simulink model "PassivityBasedFinale"  (R2024b)
settings: Solver=VariableStepAuto  StartTime=0.0  StopTime=60  RelTol=1e-3
InitFcn:
  | %  Butterworth filter
  |  r=3;
  |  [b, a] = butter(r, 5, 'low', 's');  % Butterworth filter of order r
  |  K = zeros(r,1);
  |  prod = 1;
  |  for j = 1:r
  |      K(j) = a(j+1)/prod;
  |     prod = prod*K(j);
  |  end
  |  K = flip(K);
  | 
  |  intv=[];
  |  for i=1:r
  |     v(i).vec = zeros(6,1);
  |      intv = [intv,v(i).vec];
  |  end
values from neighbouring files (symbols this model uses):
  Ts = 0.001    [traj_genPassivity.m]
undefined symbols (not defined in the file or in its folder): dspblkCoreblockFVToolHelper, gcbh
libraries: robotcorelib x1, uavutilslib x1
settings Model: Creator=mattr  LastModifiedBy=mattr

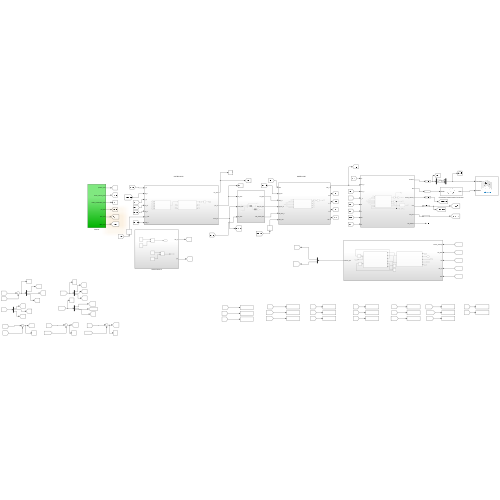
[thumbnail: Simulink's stored preview of the top-level diagram]
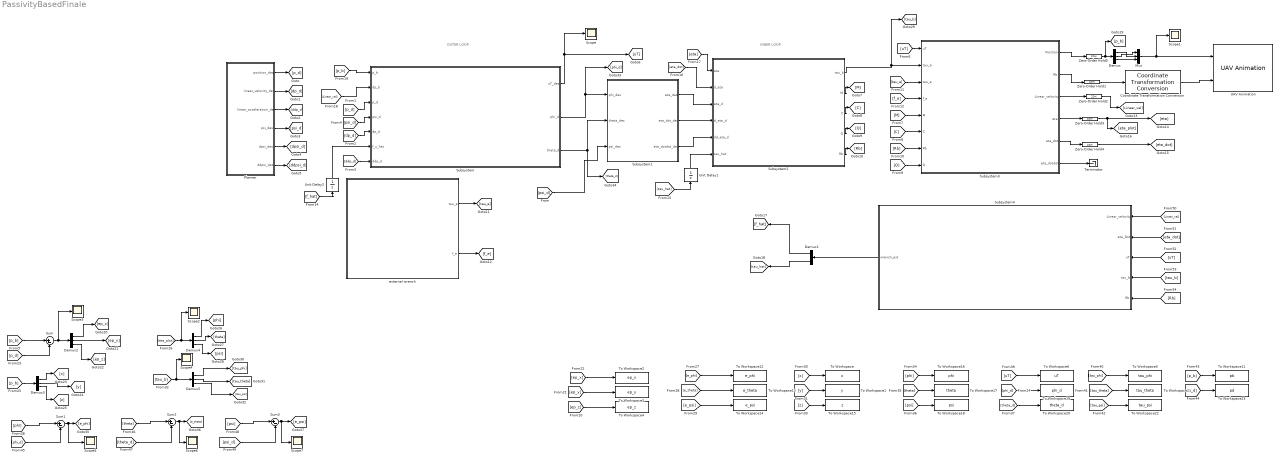
== system PassivityBasedFinale ==
  note: INNER LOOP
  note: OUTER LOOP
  Coordinate Transformation Conversion : robotcorelib/Coordinate Transformation Conversion  InputRepresentation=Rotation Matrix  InputEulerSequence=ZYX  ShowTrVecInputPort=on  OutputRepresentation=Quaternion  OutputEulerSequence=ZYX  ShowTrVecOutputPort=on  SimulateUsing=Interpreted execution
  Demux{,2..5} (5 alike) : Demux  Outputs=3
  Demux1 : Demux  Outputs=2
  Mux : Mux  Inputs=3
  Planner : Subsystem
  Scope{,1..7} (8 alike) : Scope
  Subsystem : Subsystem
  Subsystem1 : Subsystem
  Subsystem2 : Subsystem
  Subsystem3 : Subsystem
  Subsystem4 : Subsystem
  Sum{,1..3} (4 alike) : Sum  Inputs=|+-
  Terminator : Terminator
  To Workspace : ToWorkspace  VariableName=x  SaveFormat=Timeseries  SampleTime=-1
  To Workspace1 : ToWorkspace  VariableName=y  SaveFormat=Timeseries  SampleTime=-1
  To Workspace11 : ToWorkspace  VariableName=pb  SaveFormat=Timeseries  SampleTime=-1
  To Workspace12 : ToWorkspace  VariableName=e_phi  SaveFormat=Timeseries  SampleTime=-1
  To Workspace13 : ToWorkspace  VariableName=e_theta  SaveFormat=Timeseries  SampleTime=-1
  To Workspace14 : ToWorkspace  VariableName=e_psi  SaveFormat=Timeseries  SampleTime=-1
  To Workspace15 : ToWorkspace  VariableName=z  SaveFormat=Timeseries  SampleTime=-1
  To Workspace16 : ToWorkspace  VariableName=phi  SaveFormat=Timeseries  SampleTime=-1
  To Workspace17 : ToWorkspace  VariableName=theta  SaveFormat=Timeseries  SampleTime=-1
  To Workspace18 : ToWorkspace  VariableName=psi  SaveFormat=Timeseries  SampleTime=-1
  To Workspace19 : ToWorkspace  VariableName=phi_d  SaveFormat=Timeseries  SampleTime=-1
  To Workspace2 : ToWorkspace  VariableName=ep_x  SaveFormat=Timeseries  SampleTime=-1
  To Workspace20 : ToWorkspace  VariableName=theta_d  SaveFormat=Timeseries  SampleTime=-1
  To Workspace21 : ToWorkspace  VariableName=tau_theta  SaveFormat=Timeseries  SampleTime=-1
  To Workspace22 : ToWorkspace  VariableName=tau_psi  SaveFormat=Timeseries  SampleTime=-1
  To Workspace23 : ToWorkspace  VariableName=pd  SaveFormat=Timeseries  SampleTime=-1
  To Workspace3 : ToWorkspace  VariableName=ep_y  SaveFormat=Timeseries  SampleTime=-1
  To Workspace4 : ToWorkspace  VariableName=ep_z  SaveFormat=Timeseries  SampleTime=-1
  To Workspace5 : ToWorkspace  VariableName=tau_phi  SaveFormat=Timeseries  SampleTime=-1
  To Workspace6 : ToWorkspace  VariableName=uT  SaveFormat=Timeseries  SampleTime=-1
  UAV Animation : uavutilslib/UAV Animation  NumUAV=1  DynamicUAVConfig=off  UAVType=Multirotor  UAVSize=1  UAVColor=[1 0 0]  UAVTrajectoryAlpha=1  InertialZDirection=Up  RotationFormat=Quaternion  DrawMarkers=off  SampleTime=-1
  Unit Delay1 : UnitDelay  InitialCondition=Ts  SampleTime=-1  HasFrameUpgradeWarning=on
  Unit Delay2 : UnitDelay  InitialCondition=Ts  SampleTime=-1  HasFrameUpgradeWarning=on
  Zero-Order Hold{1..5} (5 alike) : ZeroOrderHold  SampleTime=Ts
  external wrench : Subsystem
  wires:
  Planner/1(position_des) -> [p_d]
  [p_d] -> Subsystem/3(p_d)
  Planner/2(linear_velocity_des) -> [dp_d]
  [dp_d] -> Subsystem/5(dp_d)
  Planner/3(linear_acceleration_des) -> [ddp_d]
  [ddp_d] -> Subsystem/7(ddp_d)
  Planner/4(psi_des) -> [psi_d]
  [psi_d] -> Subsystem/4(psi_d)
  Planner/5(dpsi_des) -> [dpsi_d]
  Planner/6(ddpsi_des) -> [ddpsi_d]
  Subsystem/2(phi_d) -> Subsystem1/1(phi_des), [phi_d]
  Subsystem/3(theta_d) -> [theta_d], Subsystem1/2(theta_des)
  [psi_d] -> Subsystem1/3(psi_des)
  Subsystem1/1(eta_des) -> Subsystem2/3(eta_d)
  Subsystem1/2(eta_dot_des) -> Subsystem2/4(d_eta_d)
  Subsystem1/3(eta_dotdot_des) -> Subsystem2/5(dd_eta_d)
  [uT] -> Subsystem3/1(uT)
  Subsystem2/1(tau_b) -> [tau_b], Subsystem3/2(tau_b)
  Subsystem2/3(C) -> [C]
  Subsystem2/2(M) -> [M]
  Subsystem2/4(Q) -> [Q]
  Subsystem2/5(Rb) -> [Rb]
  [M] -> Subsystem3/5(M)
  [C] -> Subsystem3/6(C)
  [Q] -> Subsystem3/8(Q)
  [Rb] -> Subsystem3/7("Rb ")
  [tau_e] -> Subsystem3/3(tau_e)
  [f_e] -> Subsystem3/4(f_e)
  external wrench/2(f_e) -> [f_e]
  external wrench/1(tau_e) -> [tau_e]
  Zero-Order Hold1/1 -> Coordinate Transformation Conversion/1
  Coordinate Transformation Conversion/1 -> UAV Animation/2
  Subsystem3/1(Position) -> Zero-Order Hold5/1
  Zero-Order Hold5/1 -> [p_b], Demux/1
  Demux/1 -> Mux/2
  Demux/2 -> Mux/1
  Demux/3 -> Mux/3
  Mux/1 -> Scope1/1, UAV Animation/1
  Zero-Order Hold2/1 -> [Linear_vel]
  Zero-Order Hold3/1 -> [eta_plot], [eta]
  Subsystem3/6(eta_dotdot) -> Terminator/1
  Zero-Order Hold4/1 -> [eta_dot]
  Subsystem4/1(wrench_ext) -> Demux1/1
  Demux1/1 -> [f_hat]
  Demux1/2 -> [tau_hat]
  [f_hat] -> Unit Delay2/1
  [tau_hat] -> Unit Delay1/1
  Unit Delay1/1 -> Subsystem2/6(tau_hat)
  [eta] -> Subsystem2/1(eta)
  [eta_dot] -> Subsystem2/2(d_eta)
  [p_b] -> Subsystem/1(p_b)
  [Linear_vel] -> Subsystem/2(dp_b)
  [theta] -> To Workspace17/1
  [x] -> To Workspace/1
  [p_b] -> To Workspace11/1
  [ep_x] -> To Workspace2/1
  [e_psi] -> To Workspace14/1
  [ep_y] -> To Workspace3/1
  [theta_d] -> To Workspace20/1
  [psi] -> To Workspace18/1
  [tau_psi] -> To Workspace22/1
  [e_phi] -> To Workspace12/1
  [tau_theta] -> To Workspace21/1
  [p_d] -> To Workspace23/1
  [y] -> To Workspace1/1
  [z] -> To Workspace15/1
  [phi_d] -> To Workspace19/1
  [e_theta] -> To Workspace13/1
  [uT] -> To Workspace6/1
  [tau_phi] -> To Workspace5/1
  [phi] -> To Workspace16/1
  [ep_z] -> To Workspace4/1
  [p_b] -> Sum/1
  [p_d] -> Sum/2
  Sum/1 -> Scope3/1, Demux2/1
  Demux2/1 -> [ep_x]
  Demux2/2 -> [ep_y]
  Demux2/3 -> [ep_z]
  [p_b] -> Demux3/1
  Demux3/1 -> [x]
  Demux3/2 -> [y]
  Demux3/3 -> [z]
  [eta_plot] -> Scope2/1, Demux4/1
  Demux4/1 -> [phi]
  Demux4/2 -> [theta]
  Demux4/3 -> [psi]
  [tau_b] -> Scope4/1, Demux5/1
  Demux5/1 -> [tau_phi]
  Demux5/2 -> [tau_theta]
  Demux5/3 -> [tau_psi]
  [phi] -> Sum1/1
  [phi_d] -> Sum1/2
  Sum1/1 -> Scope5/1, [e_phi]
  [theta] -> Sum2/1
  [theta_d] -> Sum2/2
  Sum2/1 -> Scope6/1, [e_theta]
  Sum3/1 -> Scope7/1, [e_psi]
  [psi] -> Sum3/1
  [psi_d] -> Sum3/2
  Subsystem/1(uT_des) -> [uT], Scope/1
  [Linear_vel] -> Subsystem4/1(Linear_velocity)
  [eta_dot] -> Subsystem4/2(eta_Dot)
  [uT] -> Subsystem4/3(uT)
  [tau_b] -> Subsystem4/4(tau_b)
  [Rb] -> Subsystem4/5(Rb)
  Unit Delay2/1 -> Subsystem/6(f_u_hat)
  Subsystem3/2(Rb) -> Zero-Order Hold1/1
  Subsystem3/3(Linear_velocity) -> Zero-Order Hold2/1
  Subsystem3/4(eta) -> Zero-Order Hold3/1
  Subsystem3/5(eta_dot) -> Zero-Order Hold4/1

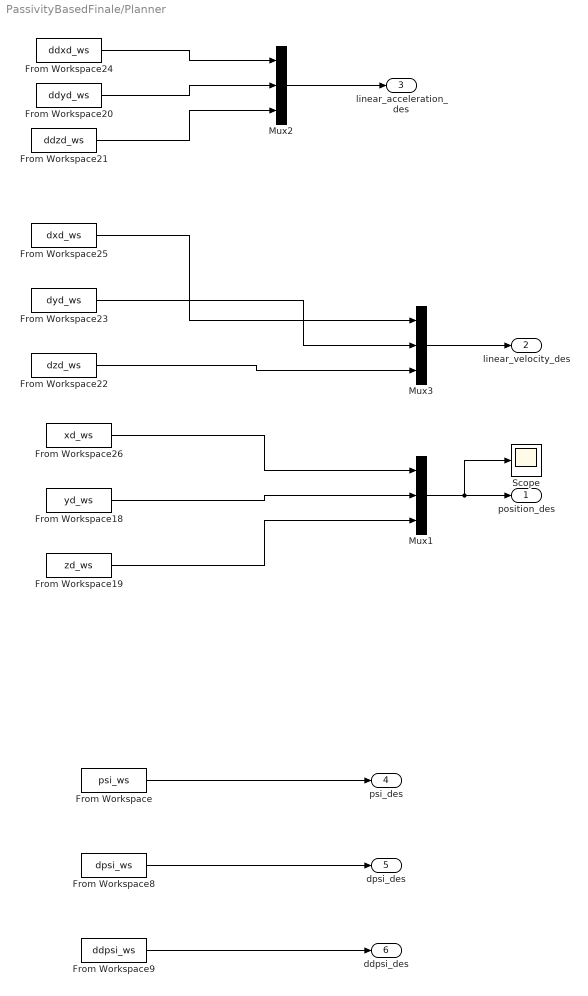
== system PassivityBasedFinale/Planner ==
  From Workspace : FromWorkspace  VariableName=psi_ws
  From Workspace18 : FromWorkspace  VariableName=yd_ws
  From Workspace19 : FromWorkspace  VariableName=zd_ws
  From Workspace20 : FromWorkspace  VariableName=ddyd_ws
  From Workspace21 : FromWorkspace  VariableName=ddzd_ws
  From Workspace22 : FromWorkspace  VariableName=dzd_ws
  From Workspace23 : FromWorkspace  VariableName=dyd_ws
  From Workspace24 : FromWorkspace  VariableName=ddxd_ws
  From Workspace25 : FromWorkspace  VariableName=dxd_ws
  From Workspace26 : FromWorkspace  VariableName=xd_ws
  From Workspace8 : FromWorkspace  VariableName=dpsi_ws
  From Workspace9 : FromWorkspace  VariableName=ddpsi_ws
  Mux1 : Mux  Inputs=3
  Mux2 : Mux  Inputs=3
  Mux3 : Mux  Inputs=3
  Scope : Scope
  position_des : Outport
  linear_velocity_des : Outport  Port=2
  linear_acceleration_des : Outport  Port=3
  psi_des : Outport  Port=4
  dpsi_des : Outport  Port=5
  ddpsi_des : Outport  Port=6
  wires:
  Mux2/1 -> linear_acceleration_des/1
  Mux1/1 -> Scope/1, position_des/1
  Mux3/1 -> linear_velocity_des/1
  From Workspace26/1 -> Mux1/1
  From Workspace18/1 -> Mux1/2
  From Workspace19/1 -> Mux1/3
  From Workspace25/1 -> Mux3/1
  From Workspace23/1 -> Mux3/2
  From Workspace22/1 -> Mux3/3
  From Workspace24/1 -> Mux2/1
  From Workspace20/1 -> Mux2/2
  From Workspace21/1 -> Mux2/3
  From Workspace/1 -> psi_des/1
  From Workspace8/1 -> dpsi_des/1
  From Workspace9/1 -> ddpsi_des/1

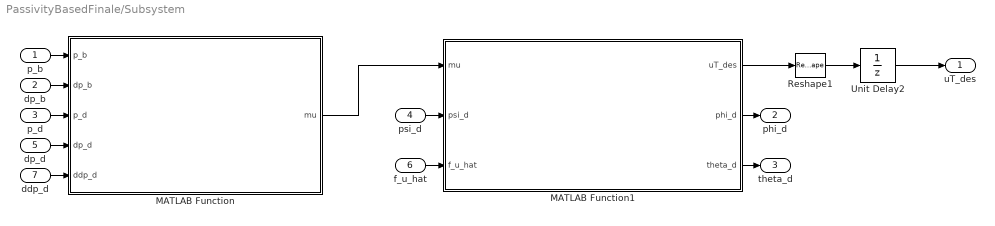
== system PassivityBasedFinale/Subsystem ==
  p_b : Inport
  dp_b : Inport  Port=2
  p_d : Inport  Port=3
  psi_d : Inport  Port=4
  dp_d : Inport  Port=5
  f_u_hat : Inport  Port=6
  ddp_d : Inport  Port=7
  MATLAB Function : MATLAB Function  TreatAsAtomicUnit=on
  MATLAB Function1 : MATLAB Function  TreatAsAtomicUnit=on
  Reshape1 : Reshape
  Unit Delay2 : UnitDelay  InitialCondition=12  SampleTime=Ts  HasFrameUpgradeWarning=on
  uT_des : Outport
  phi_d : Outport  Port=2
  theta_d : Outport  Port=3
  wires:
  p_b/1 -> MATLAB Function/1(p_b)
  psi_d/1 -> MATLAB Function1/2(psi_d)
  ddp_d/1 -> MATLAB Function/5(ddp_d)
  f_u_hat/1 -> MATLAB Function1/3(f_u_hat)
  dp_d/1 -> MATLAB Function/4(dp_d)
  dp_b/1 -> MATLAB Function/2(dp_b)
  p_d/1 -> MATLAB Function/3(p_d)
  MATLAB Function1/2(phi_d) -> phi_d/1
  MATLAB Function1/3(theta_d) -> theta_d/1
  MATLAB Function1/1(uT_des) -> Reshape1/1
  Reshape1/1 -> Unit Delay2/1
  Unit Delay2/1 -> uT_des/1
  MATLAB Function/1(mu) -> MATLAB Function1/1(mu)

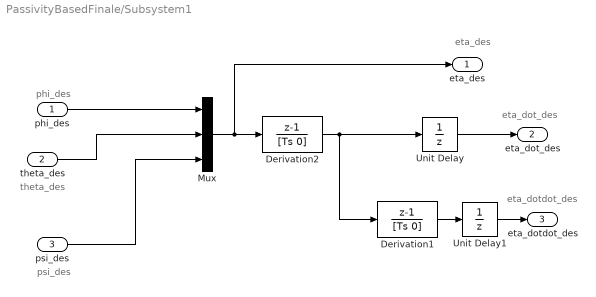
== system PassivityBasedFinale/Subsystem1 ==
  note: eta_dotdot_des
  note: eta_dot_des
  note: eta_des
  note: theta_des
  note: psi_des
  note: phi_des
  phi_des : Inport
  theta_des : Inport  Port=2
  psi_des : Inport  Port=3
  Derivation1 : DiscreteTransferFcn  LoadFcn=dspblkCoreblockFVToolHelper(gcbh,'load');  Numerator=[1 -1]  Denominator=[Ts 0]  InitialStates=[0 0 0]  SampleTime=Ts
      settings: CopyFcn=dspblkCoreblockFVToolHelper(gcbh,'copy');  DeleteFcn=dspblkCoreblockFVToolHelper(gcbh,'close');  ModelCloseFcn=dspblkCoreblockFVToolHelper(gcbh,'close');  PreSaveFcn=dspblkCoreblockFVToolHelper(gcbh,'presave');  PostSaveFcn=dspblkCoreblockFVToolHelper(gcbh,'postsave');  CloseFcn=dspblkCoreblockFVToolHelper(gcbh,'close');
  Derivation2 : DiscreteTransferFcn  LoadFcn=dspblkCoreblockFVToolHelper(gcbh,'load');  Numerator=[1 -1]  Denominator=[Ts 0]  InitialStates=[0 0 0]  SampleTime=Ts
      settings: CopyFcn=dspblkCoreblockFVToolHelper(gcbh,'copy');  DeleteFcn=dspblkCoreblockFVToolHelper(gcbh,'close');  ModelCloseFcn=dspblkCoreblockFVToolHelper(gcbh,'close');  PreSaveFcn=dspblkCoreblockFVToolHelper(gcbh,'presave');  PostSaveFcn=dspblkCoreblockFVToolHelper(gcbh,'postsave');  CloseFcn=dspblkCoreblockFVToolHelper(gcbh,'close');
  Mux : Mux  Inputs=3
  Unit Delay : UnitDelay  InitialCondition=[0 0 0]  SampleTime=-1  HasFrameUpgradeWarning=on
  Unit Delay1 : UnitDelay  InitialCondition=[0 0 0]  SampleTime=-1  HasFrameUpgradeWarning=on
  eta_des : Outport
  eta_dot_des : Outport  Port=2
  eta_dotdot_des : Outport  Port=3
  wires:
  psi_des/1 -> Mux/3
  theta_des/1 -> Mux/2
  phi_des/1 -> Mux/1
  Mux/1 -> Derivation2/1, eta_des/1
  Derivation2/1 -> Derivation1/1, Unit Delay/1
  Unit Delay/1 -> eta_dot_des/1
  Derivation1/1 -> Unit Delay1/1
  Unit Delay1/1 -> eta_dotdot_des/1

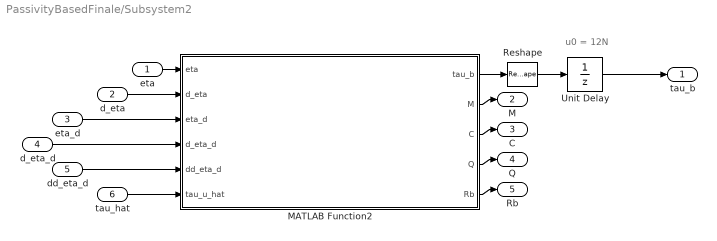
== system PassivityBasedFinale/Subsystem2 ==
  note: u0 = 12N
  eta : Inport
  d_eta : Inport  Port=2
  eta_d : Inport  Port=3
  d_eta_d : Inport  Port=4
  dd_eta_d : Inport  Port=5
  tau_hat : Inport  Port=6
  MATLAB Function2 : MATLAB Function  TreatAsAtomicUnit=on
  Reshape : Reshape
  Unit Delay : UnitDelay  InitialCondition=12  SampleTime=Ts  HasFrameUpgradeWarning=on
  tau_b : Outport
  M : Outport  Port=2
  C : Outport  Port=3
  Q : Outport  Port=4
  Rb : Outport  Port=5
  wires:
  d_eta/1 -> MATLAB Function2/2(d_eta)
  MATLAB Function2/4(Q) -> Q/1
  MATLAB Function2/3(C) -> C/1
  d_eta_d/1 -> MATLAB Function2/4(d_eta_d)
  dd_eta_d/1 -> MATLAB Function2/5(dd_eta_d)
  eta/1 -> MATLAB Function2/1(eta)
  MATLAB Function2/2(M) -> M/1
  eta_d/1 -> MATLAB Function2/3(eta_d)
  MATLAB Function2/5(Rb) -> Rb/1
  tau_hat/1 -> MATLAB Function2/6(tau_u_hat)
  Reshape/1 -> Unit Delay/1
  MATLAB Function2/1(tau_b) -> Reshape/1
  Unit Delay/1 -> tau_b/1

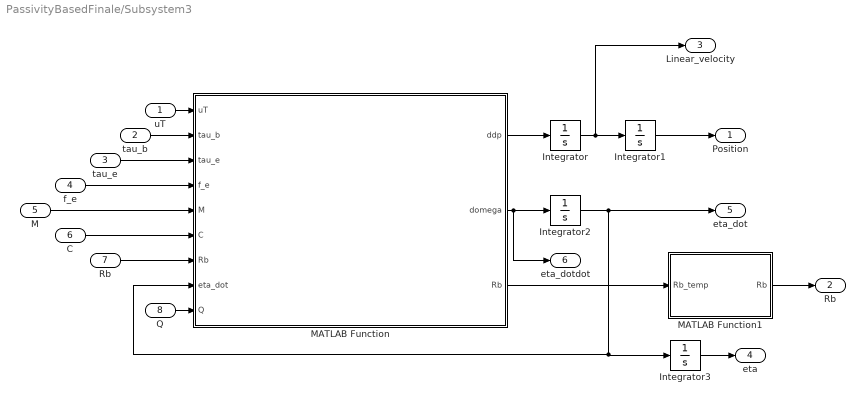
== system PassivityBasedFinale/Subsystem3 ==
  uT : Inport
  tau_b : Inport  Port=2
  tau_e : Inport  Port=3
  f_e : Inport  Port=4
  M : Inport  Port=5
  C : Inport  Port=6
  "Rb " : Inport  Port=7
  Q : Inport  Port=8
  Integrator : Integrator  InitialCondition=|
      | [ -9.8696e-05, 
      |     0.6283
      | ,    3.3333e-06]
  Integrator1 : Integrator  InitialCondition=[0 0 0]
  Integrator2 : Integrator  InitialCondition=[0 0 0]'
  Integrator3 : Integrator  InitialCondition=[0 0 0]'
  MATLAB Function : MATLAB Function  TreatAsAtomicUnit=on
  MATLAB Function1 : MATLAB Function  TreatAsAtomicUnit=on
  Position : Outport
  Rb : Outport  Port=2
  Linear_velocity : Outport  Port=3
  eta : Outport  Port=4
  eta_dot : Outport  Port=5
  eta_dotdot : Outport  Port=6
  wires:
  C/1 -> MATLAB Function/6(C)
  "Rb "/1 -> MATLAB Function/7("Rb ")
  tau_e/1 -> MATLAB Function/3(tau_e)
  tau_b/1 -> MATLAB Function/2(tau_b)
  f_e/1 -> MATLAB Function/4(f_e)
  uT/1 -> MATLAB Function/1(uT)
  M/1 -> MATLAB Function/5(M)
  Q/1 -> MATLAB Function/9(Q)
  MATLAB Function/3(Rb) -> MATLAB Function1/1(Rb_temp)
  MATLAB Function/1(ddp) -> Integrator/1
  Integrator/1 -> Linear_velocity/1, Integrator1/1
  Integrator1/1 -> Position/1
  MATLAB Function/2(domega) -> eta_dotdot/1, Integrator2/1
  Integrator2/1 -> MATLAB Function/8(eta_dot), Integrator3/1, eta_dot/1
  MATLAB Function1/1(Rb) -> Rb/1
  Integrator3/1 -> eta/1

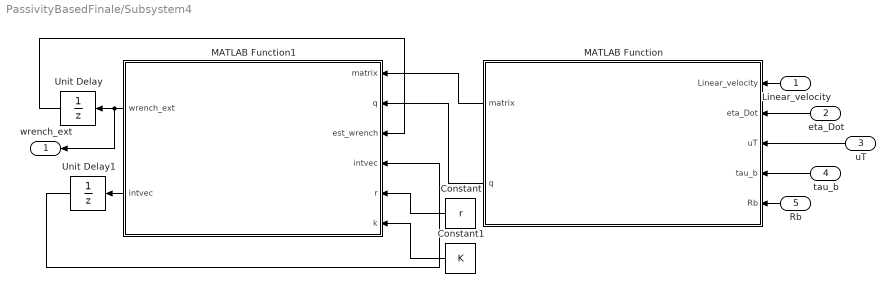
== system PassivityBasedFinale/Subsystem4 ==
  Linear_velocity : Inport
  eta_Dot : Inport  Port=2
  uT : Inport  Port=3
  tau_b : Inport  Port=4
  Rb : Inport  Port=5
  Constant : Constant  Value=r
  Constant1 : Constant  Value=K
  MATLAB Function : MATLAB Function  TreatAsAtomicUnit=on
  MATLAB Function1 : MATLAB Function  TreatAsAtomicUnit=on
  Unit Delay : UnitDelay  InitialCondition=zeros(6,1)  SampleTime=Ts  HasFrameUpgradeWarning=on
  Unit Delay1 : UnitDelay  InitialCondition=intv  SampleTime=Ts  HasFrameUpgradeWarning=on
  wrench_ext : Outport
  wires:
  Constant/1 -> MATLAB Function1/5(r)
  Unit Delay1/1 -> MATLAB Function1/4("intvec ")
  MATLAB Function1/2(intvec) -> Unit Delay1/1
  MATLAB Function/2(q) -> MATLAB Function1/2(q)
  Linear_velocity/1 -> MATLAB Function/1(Linear_velocity)
  tau_b/1 -> MATLAB Function/4(tau_b)
  uT/1 -> MATLAB Function/3(uT)
  Rb/1 -> MATLAB Function/5(Rb)
  eta_Dot/1 -> MATLAB Function/2(eta_Dot)
  MATLAB Function/1(matrix) -> MATLAB Function1/1(matrix)
  Unit Delay/1 -> MATLAB Function1/3(est_wrench)
  Constant1/1 -> MATLAB Function1/6(k)
  MATLAB Function1/1(wrench_ext) -> wrench_ext/1, Unit Delay/1

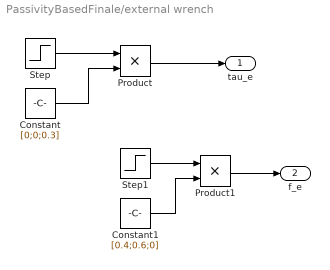
== system PassivityBasedFinale/external wrench ==
  Constant : Constant  Value=[0;0;0.3]  SampleTime=Ts
  Constant1 : Constant  Value=[0.4;0.6;0]  SampleTime=Ts
  Product : Product
  Product1 : Product
  Step : Step  Time=12  SampleTime=Ts
  Step1 : Step  Time=12  SampleTime=Ts
  tau_e : Outport
  f_e : Outport  Port=2
  wires:
  Step1/1 -> Product1/1
  Constant/1 -> Product/2
  Constant1/1 -> Product1/2
  Step/1 -> Product/1
  Product1/1 -> f_e/1
  Product/1 -> tau_e/1

== matlab function PassivityBasedFinale/Subsystem/MATLAB Function1 ==
  data: mu input; uT_des output; psi_d input; f_u_hat input; phi_d output; theta_d output
function [uT_des, phi_d,theta_d] = thrust_attitude_ref(mu, psi_d, f_u_hat)
% === PARAMETERS ===
m = 1.8;
g = 9.81;

mu_bar = mu - (1/m) * f_u_hat;
mu1 = mu_bar(1);
mu2 = mu_bar(2);
mu3 = mu_bar(3);

% === THRUST ===
uT_des = m * sqrt(mu1^2 + mu2^2 + (mu3 - g)^2);

% === DESIRED ANGLES ===
phi_arg = (m/uT_des)*(mu2 * cos(psi_d) - mu1 * sin(psi_d));
phi_d = asin(phi_arg);
theta_d = atan((mu1 * cos(psi_d) + mu2 * sin(psi_d))/(mu3 - g));
end

== matlab function PassivityBasedFinale/Subsystem/MATLAB Function ==
  data: p_b input; mu output; dp_b input; p_d input; dp_d input; ddp_d input
function mu = position_passive_control(p_b, dp_b, ...
                                        p_d, dp_d, ddp_d)
m = 1.8;

Kp = diag([25, 25, 10]);
Dp = diag([10, 10, 20]);

e_p = p_b - p_d;
de_p = dp_b - dp_d;

mu = ddp_d - (1/m)*(Dp*de_p + Kp*e_p);
end

== matlab function PassivityBasedFinale/Subsystem2/MATLAB Function2 ==
  data: eta input; tau_b output; d_eta input; eta_d input; d_eta_d input; dd_eta_d input; M output; C output; Q output; Rb output; tau_u_hat input
function [tau_b, M,C,Q,Rb] = attitude_passive_control(eta, d_eta, ...
    eta_d, d_eta_d, dd_eta_d, ...
    tau_u_hat)
% === PARAMETERS ===
Ko = diag([36, 36, 90]);
Do = diag([4, 4, 16]);
nu = 2; % Coupling parameter 

% Drone inertia
I = diag([0.035, 0.035, 0.05]); % Inertia matrix [kg·m²]

% === TRACKING ERRORS ===
e_eta = eta - eta_d; % angular position error
de_eta = d_eta - d_eta_d; % angular velocity error

% === REFERENCE VELOCITY  ===
d_eta_r = d_eta_d - nu * e_eta; % η̇_r = η̇_d - ν*e_η

% === REFERENCE ACCELERATION ===
dd_eta_r = dd_eta_d - nu * de_eta; % η̈_r = η̈_d - ν*ė_η

% === VELOCITY ERROR v_η  ===
v_eta = de_eta + nu * e_eta; % v_η = ė_η + ν*e_η


phi = eta(1);
theta = eta(2);
psi = eta(3);

c_phi = cos(phi); s_phi = sin(phi);
c_theta = cos(theta); s_theta = sin(theta);

Q = [1, 0, -s_theta;
     0, c_phi, s_phi*c_theta;
     0, -s_phi, c_phi*c_theta];

M = Q' * I * Q;

dphi = d_eta(1);
dtheta = d_eta(2);
dpsi = d_eta(3);

dQ = [0, 0, -c_theta*dtheta;
      0, -s_phi*dphi, c_phi*c_theta*dphi - s_phi*s_theta*dtheta;
      0, -c_phi*dphi, +s_phi*c_theta*dphi - c_phi*s_theta*dtheta];

omega_b = Q * d_eta; % angular velocity in body frame
S_omega_b = skew(omega_b);
C = Q' * S_omega_b * I * Q + Q' * I * dQ;

Rb = [cos(psi)*cos(theta), -sin(psi)*cos(phi)+cos(psi)*sin(theta)*sin(phi), sin(psi)*sin(phi)+cos(psi)*sin(theta)*cos(phi);
      sin(psi)*cos(theta), cos(psi)*cos(phi)+sin(psi)*sin(theta)*sin(phi), -cos(psi)*sin(phi)+sin(psi)*sin(theta)*cos(phi);
      -sin(theta), cos(theta)*sin(phi), cos(theta)*cos(phi)];

% Controller term
control_term = M * dd_eta_r + C * d_eta_r - Do * v_eta - Ko * e_eta - tau_u_hat;
tau_b = Q' \ control_term;
end

% === SKEW MATRIX ===
function S = skew(v)
if length(v) == 3
    S = [ 0   -v(3)  v(2);
         v(3)   0   -v(1);
        -v(2)  v(1)   0  ];
else
    S = zeros(3,3);
end
end

== matlab function PassivityBasedFinale/Subsystem3/MATLAB Function ==
  data: uT input; ddp output; tau_b input; tau_e input; f_e input; M input; C input; Rb input; eta_dot input; Q input; domega output; Rb output
function [ddp,domega,Rb]=vtol_uav(uT,tau_b,tau_e,f_e,M,C,Rb,eta_dot,Q)
% === PARAMETERS ===
mass = 1.8; % mass [kg]
g = 9.81; % gravity [m/s²]


% === TRANSLATIONAL DYNAMICS ===
ddp = 9.81*[0 0 1]' - (uT/mass)*Rb*[0 0 1]' + (1/mass)*f_e;

% === ROTATIONAL DYNAMICS ===
domega = M\(-C*eta_dot + Q'*tau_b + tau_e);
end

== matlab function PassivityBasedFinale/Subsystem3/MATLAB Function1 ==
  data: Rb_temp input; Rb output
function Rb = fcn(Rb_temp)
    [U,S,V] = svd(Rb_temp);
    sigma = det(U*V');
    S_ = diag([1 1 sigma]);

    Rb = U*S_*V';
end

== matlab function PassivityBasedFinale/Subsystem4/MATLAB Function ==
  data: Linear_velocity input; matrix output; eta_Dot input; uT input; tau_b input; Rb input; q output
function [matrix, q] = computations(Linear_velocity, eta_Dot, uT, tau_b, Rb)
mass= 1.8; 
g = 9.81;
Ib = diag([0.035, 0.035, 0.05]);
q = [mass*eye(3) zeros(3); zeros(3) Ib] * [Linear_velocity; eta_Dot];  
matrix = [mass*g*[0 0 1]'-uT*Rb*[0 0 1]'; -skew(eta_Dot)*Ib*eta_Dot + tau_b];
end

function S = skew(v)
if(numel(v)~= 1)
S= [0 -v(3) v(2); 
    v(3) 0 -v(1);
    -v(2) v(1) 0];
else
S= zeros(3);
end
end

== matlab function PassivityBasedFinale/Subsystem4/MATLAB Function1 ==
  data: matrix input; wrench_ext output; q input; est_wrench input; intvec input; r input; k input; intvec output
function [wrench_ext,intvec] = estimation(matrix,q,est_wrench,intvec,r,k)

    dt=1e-3;
    gamma=zeros(6,r);

    for i=1:r
        if i==1
            intvec(:,i) = intvec(:,i) + (est_wrench+matrix)*dt;
            gamma(:,i) = k(i)*(q-intvec(:,i));
        else
            intvec(:,i) = intvec(:,i) + (-est_wrench+gamma(:,i-1))*dt;
            gamma(:,i) = k(i)*intvec(:,i);
        end
    end
    wrench_ext = gamma(:,r);

end
